simulink model "gtm_design_lpv"  (R2021b)
settings: Solver=VariableStepAuto  StartTime=0.0  StopTime=10  FixedStep=0.005  MaxStep=0.005  RelTol=1e-3
StopFcn:
  | MWSout=grabmws(bdroot);
  | MWSout.lastrun=datestr(now);
values from neighbouring files (symbols this model uses):
  s = tf('s')    [SingleDOF.m]    (also in main.m; mainSimple.m; newmain.m)
undefined symbols (not defined in the file or in its folder): Aero, aftfuel, aftfuel_pos, AILL, AILLC, AILR, AILRC, alpha_deg, altitude_ft, Ax_g, Ay_g, Az_g, b, beta_deg, bias, BRAKEC, Cbar, cg_pos0, cg_shift_gear, DamageCase, DamageModels, DamageOnsetTime, Earth, ELLIB, ELLIBC, ELLOB, ELLOBC, ELRIB, ELRIBC, ELROB, ELROBC, engl_ang, engl_pos, engr_ang, engr_pos, FLAPLIB, FLAPLIC, FLAPLOB, FLAPLOC, FLAPRIB, FLAPRIC, FLAPROB, FLAPROC, ft, FuelUsed_Init, fwdfuel, fwdfuel_pos, GEAR, GEARC, Inertia0, Inertia_shift_gear, Ixx_model, Iyy_model, Izz_model, KTAS, LandingGear, LengON, LinearizeModeOn, NAV_altitude_m, NAV_latitude_deg ... (+51)
libraries: simulink_extras x63, simulink_need_slupdate x30, LPVBlockLibrary x20, aerolibconvert2 x6, aerolibtransform2 x5, uavalgslib x4, UserContent_lib x3, simulink x3, robotcorelib x1, uavutilslib x1
(part 1 of 8)
settings Model: LastModifiedBy=jihoo
settings DataIOCC: ReturnWorkspaceOutputs=off
settings OptimizationCC: BlockReduction=off  BooleanDataType=off
settings DebuggingCC: SaveWithParameterizedLinksMsg=none  UnderspecifiedInitializationDetection=Classic  MergeDetectMultiDrivingBlocksExec=none  SignalResolutionControl=TryResolveAllWithWarning  InitInArrayFormatMsg=none
settings HardwareCC: TargetUnknown=on
settings ModelReferenceCC: PropagateSignalLabelsOutOfModel=off

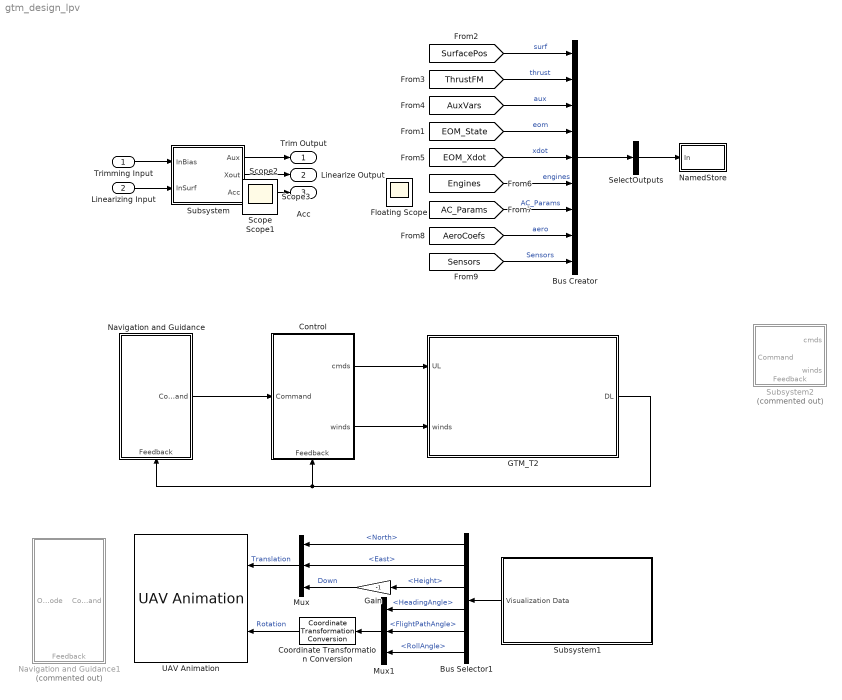
== system gtm_design_lpv ==
  Trimming Input : Inport  OutDataTypeStr=double  PortDimensions=4
  Linearizing Input : Inport  Port=2  OutDataTypeStr=double  PortDimensions=19
  Bus Creator : BusCreator  Inputs=9
  Bus Selector1 : BusSelector  OutputSignals=North,East,Height,HeadingAngle,FlightPathAngle,RollAngle
  Control : Subsystem
      settings: PortSchema="{\"entries\":[{\"content\":{\"sides\":[{\"content\":{\"connectorIds\":[\"In1\"]},\"type\":\"ConnectorPlacement.EquallySpacedRectSide\",\"uuid\":\"876f9d1c-31d1-4d48-8cbb-f6088518770e\"},{\"content\":{\"connectorIds\":[\"Out1\",\"Out2\"],\"side\":\"RIGHT\"},\"type\":\"ConnectorPlacement.EquallySpacedRectSide\",\"uuid\":\"0e4266e3-a031-465f-8381-066e8420e2a4\"},{\"content\":{\"connectorIds\":[],\"side\":\"TOP\"},\"type\":\"ConnectorPlacement.EquallySpacedRectSide\",\"uuid\":\"3957ab9c-ff96-432b-bd6f-14b7cf2f8092\"},{\"content\":{\"connectorIds\":[\"In2\"],\"side\":\"BOTTOM\"},\"type\":\"ConnectorPlacement.EquallySpacedRectSide\",\"uuid\":\"1e447cfa-7c82-4ae0-9a3c-28fe1a02d81e\"}]},\"type\":\"ConnectorPlacement.EquallySpacedConnector\",\"uuid\":\"5c345d19-69a3-46c5-b9cf-f35f763eae5c\"}],\"packageUris\":[\"http://schema.mathworks.com/mf0/Connector/R2020b\"],\"version\":\"1.0\"}"
  Coordinate Transformation Conversion : robotcorelib/Coordinate Transformation Conversion  InputRepresentation=Euler Angles  InputEulerSequence=ZYX  ShowTrVecInputPort=on  OutputRepresentation=Quaternion  OutputEulerSequence=ZYX  ShowTrVecOutputPort=on  SimulateUsing=Code generation
      settings: SourceProductBaseCode=NV,RO,RR,UV
  GTM_T2 : Subsystem  Tag=From trunk/GTMsim/gtm_model.mdl revision 162
      mask Display: image(imread('GTMtiny.png'))
  Gain : Gain  Gain=-1
  Mux : Mux  Inputs=3
  Mux1 : Mux  Inputs=3
  NamedStore : Subsystem  StopFcn=|  mask{enable_logging=on, do_stopfcn_callback=on}
      | % if strmatch(get_param(gcb,'do_stopfcn_callback'),...
      | % 'on','exact')                                       
      | %    if exist('logsout','var')                        
      | %        sout = CreateSimOut(logsout);                
      | %    else                                             
      | %         %disp('No Log Data Variable')               
      | %     end                                             
      | % clear logsout                                       
      | % end
      mask prompts: enable_logging "Enable Data Logging"; do_stopfcn_callback "Post-process logsout"
      mask help: Produces signal log of input data. If post processing is selected the logsout object is converted into a data structure (sout) with fields named after the bus signals. In this case a common time base is recommended.
      mask init:
      | H=get_param([gcb,'/In'],'PortHandles');
      | if (enable_logging)
      |     set(H.Outport(1),'DataLogging','on')
      | else
      |     set(H.Outport(1),'DataLogging','off')
      |     
      | end
  Navigation and Guidance : Subsystem
      settings: PortSchema="{\"entries\":[{\"content\":{\"sides\":[{\"content\":{\"connectorIds\":[]},\"type\":\"ConnectorPlacement.EquallySpacedRectSide\",\"uuid\":\"90854f57-5bb3-4250-804d-ac09ea809a44\"},{\"content\":{\"connectorIds\":[\"Out1\"],\"side\":\"RIGHT\"},\"type\":\"ConnectorPlacement.EquallySpacedRectSide\",\"uuid\":\"60962e56-1ad7-44d3-901b-e4e8a3eb3ce1\"},{\"content\":{\"connectorIds\":[],\"side\":\"TOP\"},\"type\":\"ConnectorPlacement.EquallySpacedRectSide\",\"uuid\":\"face4b20-fd55-46eb-98c2-63599aba0959\"},{\"content\":{\"connectorIds\":[\"In1\"],\"side\":\"BOTTOM\"},\"type\":\"ConnectorPlacement.EquallySpacedRectSide\",\"uuid\":\"a5d6b840-59da-4fbb-8659-3c66a691c6e0\"}]},\"type\":\"ConnectorPlacement.EquallySpacedConnector\",\"uuid\":\"30f94791-aa21-40a3-94e2-49d0efe50b10\"}],\"packageUris\":[\"http://schema.mathworks.com/mf0/Connector/R2020b\"],\"version\":\"1.0\"}"
  Navigation and Guidance1 : Subsystem  Commented=on
      settings: PortSchema="{\"entries\":[{\"content\":{\"sides\":[{\"content\":{\"connectorIds\":[\"In1\"]},\"type\":\"ConnectorPlacement.EquallySpacedRectSide\",\"uuid\":\"90854f57-5bb3-4250-804d-ac09ea809a44\"},{\"content\":{\"connectorIds\":[\"Out1\"],\"side\":\"RIGHT\"},\"type\":\"ConnectorPlacement.EquallySpacedRectSide\",\"uuid\":\"60962e56-1ad7-44d3-901b-e4e8a3eb3ce1\"},{\"content\":{\"connectorIds\":[],\"side\":\"TOP\"},\"type\":\"ConnectorPlacement.EquallySpacedRectSide\",\"uuid\":\"face4b20-fd55-46eb-98c2-63599aba0959\"},{\"content\":{\"connectorIds\":[\"In2\"],\"side\":\"BOTTOM\"},\"type\":\"ConnectorPlacement.EquallySpacedRectSide\",\"uuid\":\"a5d6b840-59da-4fbb-8659-3c66a691c6e0\"}]},\"type\":\"ConnectorPlacement.EquallySpacedConnector\",\"uuid\":\"30f94791-aa21-40a3-94e2-49d0efe50b10\"}],\"packageUris\":[\"http://schema.mathworks.com/mf0/Connector/R2020b\"],\"version\":\"1.0\"}"
  SelectOutputs : BusSelector  OutputSignals=surf,thrust,aux,eom,xdot,engines,AC_Params,aero,Sensors  OutputAsBus=on
  Subsystem : Subsystem
  Subsystem1 : Subsystem
  Subsystem2 : Subsystem  Commented=on
      settings: PortSchema="{\"entries\":[{\"content\":{\"sides\":[{\"content\":{\"connectorIds\":[\"In1\"]},\"type\":\"ConnectorPlacement.EquallySpacedRectSide\",\"uuid\":\"5c2295be-4c8d-43d5-89d0-a9519d1e786b\"},{\"content\":{\"connectorIds\":[\"Out1\",\"Out2\"],\"side\":\"RIGHT\"},\"type\":\"ConnectorPlacement.EquallySpacedRectSide\",\"uuid\":\"0338c219-9523-4a98-a604-936e4d0799a1\"},{\"content\":{\"connectorIds\":[],\"side\":\"TOP\"},\"type\":\"ConnectorPlacement.EquallySpacedRectSide\",\"uuid\":\"01cfcb74-d03a-4fe9-8f17-a2d3b8ee66f0\"},{\"content\":{\"connectorIds\":[\"In2\"],\"side\":\"BOTTOM\"},\"type\":\"ConnectorPlacement.EquallySpacedRectSide\",\"uuid\":\"93f21525-f5cf-4ae2-b844-2a7328abed77\"}]},\"type\":\"ConnectorPlacement.EquallySpacedConnector\",\"uuid\":\"4d608291-8d9a-4652-b4af-32d3e417625b\"}],\"packageUris\":[\"http://schema.mathworks.com/mf0/Connector/R2020b\"],\"version\":\"1.0\"}"
  UAV Animation : uavutilslib/UAV Animation  UAVType=FixedWing  UAVSize=50  InertialZDirection=Down  SampleTime=0.1
      settings: SourceProductBaseCode=UV
  Trim Output : Outport  OutDataTypeStr=double  PortDimensions=6
  Linearize Output : Outport  Port=2  OutDataTypeStr=double  PortDimensions=12
  Acc : Outport  Port=3  OutDataTypeStr=double  PortDimensions=3
  Floating Scope : Scope
  Scope{,1..3} (4 alike) : Scope
  wires:
  Linearizing Input/1 -> Subsystem/2(InSurf)
  Subsystem/1(Aux) -> Trim Output/1
  Subsystem/2(Xout) -> Linearize Output/1
  Trimming Input/1 -> Subsystem/1(InBias)
  Control/1(cmds) -> GTM_T2/1(UL)
  Control/2(winds) -> GTM_T2/2(winds)
  Subsystem/3(Acc) -> Acc/1
  Bus Selector1/6 -> Mux1/3  "<RollAngle>"
  Mux/1 -> UAV Animation/1  "Translation"
  Bus Selector1/2 -> Mux/2  "<East>"
  Mux1/1 -> Coordinate Transformation Conversion/1
  Bus Selector1/1 -> Mux/1  "<North>"
  Bus Selector1/4 -> Mux1/1  "<HeadingAngle>"
  Coordinate Transformation Conversion/1 -> UAV Animation/2  "Rotation"
  Bus Selector1/3 -> Gain/1  "<Height>"
  Bus Selector1/5 -> Mux1/2  "<FlightPathAngle>"
  Gain/1 -> Mux/3  "Down"
  GTM_T2/1(DL) -> Navigation and Guidance/1(Feedback), Control/2(Feedback)
  Navigation and Guidance/1(Command) -> Control/1(Command)
  Subsystem1/1(Visualization Data) -> Bus Selector1/1
  SelectOutputs/1 -> NamedStore/1(In)
  [AuxVars] -> Bus Creator/3  "aux"
  [ThrustFM] -> Bus Creator/2  "thrust"
  Bus Creator/1 -> SelectOutputs/1
  [SurfacePos] -> Bus Creator/1  "surf"
  [Sensors] -> Bus Creator/9  "Sensors"
  [Engines] -> Bus Creator/6  "engines"
  [EOM_Xdot] -> Bus Creator/5  "xdot"
  [AeroCoefs] -> Bus Creator/8  "aero"
  [AC_Params] -> Bus Creator/7  "AC_Params"
  [EOM_State] -> Bus Creator/4  "eom"

== system gtm_design_lpv/Control ==
  note: Input aileron command
      | +ail_cmd = roll left
  Command : Inport
  Feedback : Inport  Port=2
  Bus Creator : BusCreator  Inputs=21
  Bus Selector : BusSelector  OutputSignals=AirData.KTAS,AirData.altitude_ft
  Constant{1..4} (4 alike) : Constant  Value=0
  Demux : Demux
  Gain{1..21} (21 alike) : Gain  SaturateOnIntegerOverflow=on  OutDataTypeStr=Inherit: Same as input  ParamDataTypeStr=Inherit: Same as input
  Hinf : Subsystem  Commented=on  TreatAsAtomicUnit=on
  Input Generator : UserContent_lib/Input Generator  Commented=on  SystemSampleTime=-1  VariantActivationTime=update diagram  Latency=0  AutoFrameSizeCalculation=off
      link override Doublet Generator: timeon=[2 12 7]  pulsewidth=[0.5 0.5 0.5]  amplitude=[0 0 0]
  LPV : Subsystem  Commented=on  TreatAsAtomicUnit=on
  LPV1 : Subsystem  Commented=on  TreatAsAtomicUnit=on
  Left Roll Spoiler Schedule : Lookup  InputValues="[-20\t-11.76\t-2.36\t0\t2.36\t11.76\t20\t]"  Table=[0 0 0 0 0 9 45]  LookUpMeth=Interpolation-Use End Values
  Right Roll Spoiler Schedule : Lookup  InputValues="[-20\t-11.76\t-2.36\t0\t2.36\t11.76\t20\t]"  Table=[45 9 0 0 0 0 0]  LookUpMeth=Interpolation-Use End Values
  Scope1 : Scope  Commented=on
  Scope3 : Scope  Commented=on
  Scope4 : Scope  Commented=on
  Throttle Controller : Subsystem
  Winds : UserContent_lib/Input Generator/Winds  WindSpeed_knots=WindSpd  WindDirection_deg=WindDir  level=None
  cmds : Outport
  winds : Outport  Port=2
  wires:
  Constant1/1 -> Left Roll Spoiler Schedule/1, Right Roll Spoiler Schedule/1
  Left Roll Spoiler Schedule/1 -> Gain12/1, Gain13/1
  Gain9/1 -> Bus Creator/1  "THROTLC"
  Gain17/1 -> Bus Creator/16  "FLAPLOC"
  Gain5/1 -> Bus Creator/4  "ELLIBC"
  Gain20/1 -> Bus Creator/19  "GEARC"
  Gain11/1 -> Bus Creator/14  "SPLROBC"
  Gain8/1 -> Bus Creator/6  "ELRIBC"
  Gain13/1 -> Bus Creator/12  "SPLLOBC"
  Demux/4 -> Gain3/1, Gain4/1
  Gain1/1 -> Bus Creator/7  "AILLC"
  Demux/1 -> Gain8/1, Gain7/1, Gain5/1, Gain6/1
  Gain7/1 -> Bus Creator/5  "ELROBC"
  Gain15/1 -> Bus Creator/18  "FLAPROC"
  Constant4/1 -> Gain20/1
  Winds/1 -> winds/1
  Demux/3 -> Gain2/1
  Gain2/1 -> Bus Creator/8  "AILRC"
  Gain3/1 -> Bus Creator/9  "RUDUPC"
  Gain21/1 -> Bus Creator/21  "STEERC"
  Constant2/1 -> Gain15/1, Gain18/1, Gain17/1, Gain16/1
  Gain14/1 -> Bus Creator/13  "SPLRIBC"
  Constant3/1 -> Gain21/1, Gain19/1
  Gain6/1 -> Bus Creator/3  "ELLOBC"
  Right Roll Spoiler Schedule/1 -> Gain14/1, Gain11/1
  Gain10/1 -> Bus Creator/2  "THROTRC"
  Gain19/1 -> Bus Creator/20  "BRAKEC"
  Gain18/1 -> Bus Creator/17  "FLAPRIC"
  Gain4/1 -> Bus Creator/10  "RUDLOC"
  Bus Creator/1 -> cmds/1
  Bus Selector/2 -> Winds/2  "<altitude_ft>"
  Gain12/1 -> Bus Creator/11  "SPLLIBC"
  Gain16/1 -> Bus Creator/15  "FLAPLIC"
  Bus Selector/1 -> Winds/1  "<KTAS>"
  Throttle Controller/1(Out1) -> Gain9/1, Gain10/1
  Command/1 -> Hinf/1(Guidance), LPV1/1(Guidance), LPV/1(Guidance)
  Feedback/1 -> Bus Selector/1, LPV1/2(Feedback), Hinf/2(Feedback), LPV/2(Feedback)
  Demux/2 -> Gain1/1
  LPV/1(Out) -> Scope3/1
  LPV1/1(Out) -> Scope4/1
  Hinf/1(Out) -> Scope1/1
  ? -> Demux/1

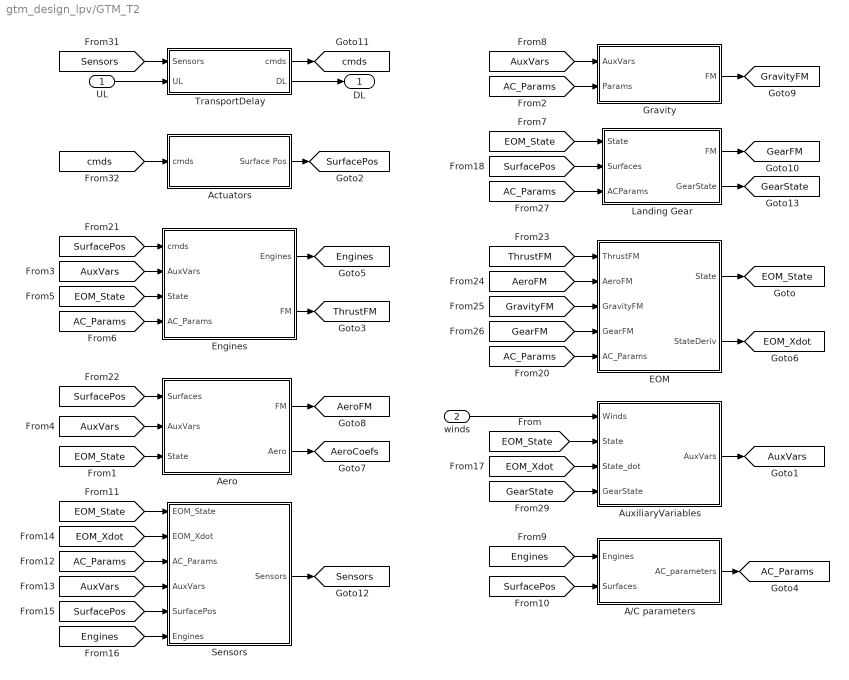
== system gtm_design_lpv/GTM_T2 ==
  UL : Inport
  winds : Inport  Port=2  PortDimensions=6
  A/C parameters : Subsystem
  Actuators : Subsystem
  Aero : Subsystem
  AuxiliaryVariables : Subsystem
  EOM : Subsystem
  Engines : Subsystem
  Gravity : Subsystem
  Landing Gear : Subsystem
  Sensors : Subsystem
  TransportDelay : Subsystem
  DL : Outport
  tag scope: AC_Params=global, AeroCoefs=global, AeroFM=global, AuxVars=global, EOM_State=global, EOM_Xdot=global, Engines=global, GearFM=global, GearState=global, GravityFM=global, Sensors=global, SurfacePos=global, ThrustFM=global, cmds=global
  wires:
  UL/1 -> TransportDelay/2(UL)
  TransportDelay/2(DL) -> DL/1
  Gravity/1(FM) -> [GravityFM]
  [AuxVars] -> Sensors/4(AuxVars)
  [EOM_Xdot] -> Sensors/2(EOM_Xdot)
  [Engines] -> Sensors/6(Engines)
  [SurfacePos] -> Sensors/5(SurfacePos)
  [AC_Params] -> Sensors/3(AC_Params)
  [EOM_State] -> Sensors/1(EOM_State)
  [AC_Params] -> EOM/5(AC_Params)
  [GearFM] -> EOM/4(GearFM)
  [GravityFM] -> EOM/3(GravityFM)
  [AeroFM] -> EOM/2(AeroFM)
  [ThrustFM] -> EOM/1(ThrustFM)
  [EOM_State] -> AuxiliaryVariables/2(State)
  [SurfacePos] -> Aero/1(Surfaces)
  [AC_Params] -> Landing Gear/3(ACParams)
  [SurfacePos] -> Engines/1(cmds)
  EOM/2(StateDeriv) -> [EOM_Xdot]
  [EOM_Xdot] -> AuxiliaryVariables/3(State_dot)
  Engines/1(Engines) -> [Engines]
  [SurfacePos] -> A/C parameters/2(Surfaces)
  [Engines] -> A/C parameters/1(Engines)
  A/C parameters/1(AC_parameters) -> [AC_Params]
  [AC_Params] -> Engines/4(AC_Params)
  [AuxVars] -> Engines/2(AuxVars)
  [EOM_State] -> Engines/3(State)
  [AuxVars] -> Gravity/1(AuxVars)
  [AC_Params] -> Gravity/2(Params)
  EOM/1(State) -> [EOM_State]
  Engines/2(FM) -> [ThrustFM]
  Aero/1(FM) -> [AeroFM]
  [AuxVars] -> Aero/2(AuxVars)
  AuxiliaryVariables/1(AuxVars) -> [AuxVars]
  [EOM_State] -> Aero/3(State)
  [EOM_State] -> Landing Gear/1(State)
  [SurfacePos] -> Landing Gear/2(Surfaces)
  Landing Gear/1(FM) -> [GearFM]
  Actuators/1(Surface Pos) -> [SurfacePos]
  winds/1 -> AuxiliaryVariables/1(Winds)
  TransportDelay/1(cmds) -> [cmds]
  [Sensors] -> TransportDelay/1(Sensors)
  [cmds] -> Actuators/1(cmds)
  Sensors/1(Sensors) -> [Sensors]
  Landing Gear/2(GearState) -> [GearState]
  [GearState] -> AuxiliaryVariables/4(GearState)
  Aero/2(Aero) -> [AeroCoefs]

== system gtm_design_lpv/NamedStore ==
  In : Inport
  Terminator : Terminator
  wires:
  In/1 -> Terminator/1  "SimOut"

== system gtm_design_lpv/Navigation and Guidance ==
  Feedback : Inport
  Bus Creator : BusCreator  Inputs=5
  Constant : Constant  Value=80
  Constant1 : Constant  Value=-12.5
  Demux : Demux  Outputs=3
  High-G Turn : Subsystem  Commented=on  TreatAsAtomicUnit=on
  Lateral Doublet : Subsystem  Commented=on  TreatAsAtomicUnit=on
  Longitudinal Doublet : Subsystem  TreatAsAtomicUnit=on
  Orbit Following : Subsystem  Commented=on  TreatAsAtomicUnit=on
  Pushover and Pullup : Subsystem  Commented=on  TreatAsAtomicUnit=on
  Scope : Scope
  Straight and Level Flight : Subsystem  Commented=on  TreatAsAtomicUnit=on
  Waypoint Following : Subsystem  Commented=on  TreatAsAtomicUnit=on
  Command : Outport
  wires:
  Bus Creator/1 -> Command/1
  Constant/1 -> Bus Creator/1  "V_c"
  Demux/1 -> Scope/1, Bus Creator/2  "An_c"
  Demux/2 -> Bus Creator/3  "beta_c"
  Demux/3 -> Bus Creator/4  "phi_c"
  Constant1/1 -> Bus Creator/5  "eta_sc"
  Feedback/1 -> Orbit Following/1(Feedback), Waypoint Following/1(Feedback)
  Longitudinal Doublet/1(Out1) -> Demux/1

== system gtm_design_lpv/Navigation and Guidance1 ==
  Operation Mode : Inport
  Feedback : Inport  Port=2
  Bus Creator : BusCreator  Inputs=5
  Constant : Constant  Value=80
  Constant1 : Constant  Value=-12.5
  Demux : Demux  Outputs=3
  High-G Turn : Subsystem  TreatAsAtomicUnit=on
  Lateral Doublet : Subsystem  TreatAsAtomicUnit=on
  Longitudinal Doublet : Subsystem  TreatAsAtomicUnit=on
  Merge : Merge  Inputs=7  InitialOutput=[1,0,0]
  Orbit Following : Subsystem  Commented=on  TreatAsAtomicUnit=on
  Pushover and Pullup : Subsystem  TreatAsAtomicUnit=on
  Straight and Level Flight : Subsystem  TreatAsAtomicUnit=on
  Switch Case2 : SwitchCase  CaseConditions={1,2,3,4,5,6}
  Waypoint Following : Subsystem  Commented=on  TreatAsAtomicUnit=on
  Command : Outport
  wires:
  Bus Creator/1 -> Command/1
  Constant/1 -> Bus Creator/1  "V_c"
  Demux/1 -> Bus Creator/2  "An_c"
  Demux/2 -> Bus Creator/3  "beta_c"
  Demux/3 -> Bus Creator/4  "phi_c"
  Constant1/1 -> Bus Creator/5  "eta_sc"
  Operation Mode/1 -> Switch Case2/1
  Feedback/1 -> Orbit Following/1(Feedback), Waypoint Following/1(Feedback)
  Longitudinal Doublet/1(Out1) -> Merge/1
  Lateral Doublet/1(Out1) -> Merge/2
  Straight and Level Flight/1(Out1) -> Merge/7
  Waypoint Following/1(Out1) -> Merge/5
  Merge/1 -> Demux/1
  Pushover and Pullup/1(Out1) -> Merge/3
  High-G Turn/1(Out1) -> Merge/4
  Orbit Following/1(Out1) -> Merge/6
  Switch Case2/1 -> Longitudinal Doublet/Action
  Switch Case2/2 -> Lateral Doublet/Action
  Switch Case2/3 -> Pushover and Pullup/Action
  Switch Case2/4 -> High-G Turn/Action
  Switch Case2/5 -> Waypoint Following/Action
  Switch Case2/6 -> Orbit Following/Action
  Switch Case2/7 -> Straight and Level Flight/Action

== system gtm_design_lpv/Subsystem ==
  InBias : Inport
  InSurf : Inport  Port=2
  Bus Selector : BusSelector  OutputSignals=eas,tas,alpha,beta,gamma,gndtrack  OutputAsBus=on
  Bus Selector1 : BusSelector  OutputSignals=Ax,Ay,Az  OutputAsBus=on
  Bus to Vector : BusToVector
  Bus to Vector1 : BusToVector
  Bus to Vector2 : BusToVector
  DocBlock : simulink/Model-Wide Utilities/DocBlock  DocumentType=Text
      content=|
      | Inputs and Outputs selected here have a specific ordering.
      |
      |
      |
      | Do not change this without also changing output channel ordering in associated linmodel.m and
      | trimgtm.m functions
  Aux : Outport
  Xout : Outport  Port=2
  Acc : Outport  Port=3
  tag scope: SurfaceBias=global, SurfaceDeltas=global
  wires:
  [EOM_State] -> Bus to Vector1/1  "eom"
  Bus Selector/1 -> Bus to Vector/1
  InSurf/1 -> [SurfaceDeltas]
  Bus to Vector/1 -> Aux/1
  Bus to Vector1/1 -> Xout/1
  InBias/1 -> [SurfaceBias]
  Bus to Vector2/1 -> Acc/1
  Bus Selector1/1 -> Bus to Vector2/1
  [AuxVars] -> Bus Selector1/1, Bus Selector/1  "aux"

== system gtm_design_lpv/Subsystem1 ==
  Bus Creator1 : BusCreator  Inputs=6
  Bus Selector1 : BusSelector  OutputSignals=latitude,longitude,altitude
  Bus Selector2 : BusSelector  OutputSignals=gndtrack,gamma
  Bus Selector3 : BusSelector  OutputSignals=phi
  Constant1 : Constant  Value=[37.827926944;-75.494061666]
  Constant2 : Constant  Value=0
  Constant3 : Constant  Value=0
  Degrees to Radians1 : simulink_extras/Transformations/Degrees to Radians
  Degrees to Radians2 : simulink_extras/Transformations/Degrees to Radians
  Demux1 : Demux  Outputs=3
      settings: DisplayOption=none
  Demux3 : Demux  Outputs=3
      settings: DisplayOption=none
  Display : Display
  Display1 : Display
  Gain : Gain  Gain=-1
  LLA to Flat Earth : aerolibtransform2/LLA to Flat Earth  units=English  ptype=Earth (WGS84)  F=1/298.257223563  R=20925646.3255  refPosPort=on  LL0=[0 10]  psi=0
      settings: SourceProductBaseCode=AE
  Mux : Mux  Inputs=3
  Mux2 : Mux  Inputs=2
  Radians to Degrees : simulink_extras/Transformations/Radians to Degrees
  Radians to Degrees1 : simulink_extras/Transformations/Radians to Degrees
  Scope : Scope
  To Workspace : ToWorkspace  VariableName=NED  SampleTime=-1
  Visualization Data : Outport
  wires:
  Demux1/3 -> Gain/1  "Down"
  Demux3/3 -> Bus Creator1/6  "RollAngle"
  Demux1/2 -> Bus Creator1/2  "East"
  Demux3/1 -> Bus Creator1/4  "HeadingAngle"
  Demux1/1 -> Bus Creator1/1  "North"
  Demux3/2 -> Bus Creator1/5  "FlightPathAngle"
  Bus Creator1/1 -> Visualization Data/1
  [EOM_State] -> Bus Selector1/1
  Gain/1 -> Bus Creator1/3  "Height"
  Bus Selector3/1 -> Mux/3  "<phi>"
  Degrees to Radians1/1 -> Mux/2  "gamma_rad"
  Degrees to Radians2/1 -> Mux/1  "gndtrack_rad"
  Mux/1 -> Demux3/1
  Constant3/1 -> LLA to Flat Earth/3
  Constant1/1 -> LLA to Flat Earth/4
  Constant2/1 -> LLA to Flat Earth/5
  Mux2/1 -> Display/1, LLA to Flat Earth/1
  Bus Selector1/3 -> Display1/1, LLA to Flat Earth/2  "<altitude>"
  [EOM_State] -> Bus Selector3/1  "eom"
  [AuxVars] -> Bus Selector2/1  "aux"
  Bus Selector2/1 -> Degrees to Radians2/1  "<gndtrack>"
  Bus Selector2/2 -> Degrees to Radians1/1  "<gamma>"
  Radians to Degrees/1 -> Mux2/1
  Radians to Degrees1/1 -> Mux2/2
  Bus Selector1/1 -> Radians to Degrees/1  "<latitude>"
  Bus Selector1/2 -> Radians to Degrees1/1  "<longitude>"
  LLA to Flat Earth/1 -> Demux1/1, To Workspace/1, Scope/1

== system gtm_design_lpv/Subsystem2 ==
  note: Input aileron command
      | +ail_cmd = roll left
  Command : Inport
  Feedback : Inport  Port=2
  Bus Creator : BusCreator  Inputs=21
  Bus Selector : BusSelector  OutputSignals=AirData.KTAS,AirData.altitude_ft
  Constant : Constant  Value=0.01
  Constant{1..4} (4 alike) : Constant  Value=0
  Demux : Demux
  Gain{1..21} (21 alike) : Gain  SaturateOnIntegerOverflow=on  OutDataTypeStr=Inherit: Same as input  ParamDataTypeStr=Inherit: Same as input
  Hinf : Subsystem  Commented=on  TreatAsAtomicUnit=on
  LPV : Subsystem  TreatAsAtomicUnit=on
  LPV1 : Subsystem  Commented=on  TreatAsAtomicUnit=on
  Left Roll Spoiler Schedule : Lookup  InputValues="[-20\t-11.76\t-2.36\t0\t2.36\t11.76\t20\t]"  Table=[0 0 0 0 0 9 45]  LookUpMeth=Interpolation-Use End Values
  Right Roll Spoiler Schedule : Lookup  InputValues="[-20\t-11.76\t-2.36\t0\t2.36\t11.76\t20\t]"  Table=[45 9 0 0 0 0 0]  LookUpMeth=Interpolation-Use End Values
  Scope1 : Scope  Commented=on
  Scope3 : Scope
  Scope4 : Scope  Commented=on
  Throttle Controller : Subsystem
  Winds : UserContent_lib/Input Generator/Winds  WindSpeed_knots=WindSpd  WindDirection_deg=WindDir  level=None
  cmds : Outport
  winds : Outport  Port=2
  wires:
  Hinf/1(Out) -> Scope1/1
  LPV/1(Out) -> Scope3/1
  LPV1/1(Out) -> Scope4/1
  Feedback/1 -> Bus Selector/1, LPV1/2(Feedback), Hinf/2(Feedback), LPV/2(Feedback)
  Winds/1 -> winds/1
  Bus Selector/1 -> Winds/1  "<KTAS>"
  Bus Selector/2 -> Winds/2  "<altitude_ft>"
  Command/1 -> Hinf/1(Guidance), LPV1/1(Guidance), LPV/1(Guidance)
  Demux/2 -> Gain1/1
  Gain21/1 -> Bus Creator/21  "STEERC"
  Gain4/1 -> Bus Creator/10  "RUDLOC"
  Demux/1 -> Gain8/1, Gain7/1, Gain5/1, Gain6/1
  Constant3/1 -> Gain21/1, Gain19/1
  Gain16/1 -> Bus Creator/15  "FLAPLIC"
  Constant2/1 -> Gain15/1, Gain18/1, Gain17/1, Gain16/1
  Gain13/1 -> Bus Creator/12  "SPLLOBC"
  Demux/3 -> Gain2/1
  Gain8/1 -> Bus Creator/6  "ELRIBC"
  Demux/4 -> Gain3/1, Gain4/1
  Gain15/1 -> Bus Creator/18  "FLAPROC"
  Gain3/1 -> Bus Creator/9  "RUDUPC"
  Gain12/1 -> Bus Creator/11  "SPLLIBC"
  Gain2/1 -> Bus Creator/8  "AILRC"
  Gain18/1 -> Bus Creator/17  "FLAPRIC"
  Gain11/1 -> Bus Creator/14  "SPLROBC"
  Right Roll Spoiler Schedule/1 -> Gain14/1, Gain11/1
  Gain17/1 -> Bus Creator/16  "FLAPLOC"
  Gain10/1 -> Bus Creator/2  "THROTRC"
  Constant4/1 -> Gain20/1
  Gain1/1 -> Bus Creator/7  "AILLC"
  Gain19/1 -> Bus Creator/20  "BRAKEC"
  Gain6/1 -> Bus Creator/3  "ELLOBC"
  Gain7/1 -> Bus Creator/5  "ELROBC"
  Gain20/1 -> Bus Creator/19  "GEARC"
  Left Roll Spoiler Schedule/1 -> Gain12/1, Gain13/1
  Constant1/1 -> Left Roll Spoiler Schedule/1, Right Roll Spoiler Schedule/1
  Gain14/1 -> Bus Creator/13  "SPLRIBC"
  Gain5/1 -> Bus Creator/4  "ELLIBC"
  Bus Creator/1 -> cmds/1
  Throttle Controller/1(Out1) -> Gain10/1, Gain9/1
  Gain9/1 -> Bus Creator/1  "THROTLC"
  Constant/1 -> Demux/1

== system gtm_design_lpv/Control/Hinf ==
  Guidance : Inport
  Feedback : Inport  Port=2
  Add : Sum
  Bus Selector : BusSelector  OutputSignals=AirData.KTAS,AirData.altitude_ft,SurfacePos.AILL,SurfacePos.AILR
  Bus Selector3 : BusSelector  OutputSignals=An_c
  Bus Selector4 : BusSelector  OutputSignals=beta_c,phi_c  OutputAsBus=on
  Bus Selector5 : BusSelector  OutputSignals=AirData.alpha_deg,MAG3.q_deg,MAG3.Az_g
  Bus Selector6 : BusSelector  OutputSignals=AirData.beta_deg,MAG3.p_deg,MAG3.r_deg,MIDG.phi_deg,MAG3.Ay_g
  Bus to Vector : BusToVector
  Bus to Vector1 : BusToVector
  Constant : Constant
  Degrees to Radians{,1..5} (6 alike) : simulink_extras/Transformations/Degrees to Radians
  Demux1 : Demux  Outputs=2
  Gain : Gain  Gain=1/2
  Gain1 : Gain  Gain=1/100
  Gain2 : Gain  Gain=32.17405
  Gain3 : Gain  Gain=32.17405
  Gain4 : Gain  Gain=100
  Gain5 : Gain  Gain=100
  LPVBlock1 : LPVBlockLibrary/LPVBlock  sys=K_lon_hinf  plist={'rho1_tas_param';'rho2_alt_param';'rho3_mor_param'}  x0=0
      settings: SourceProductName=LPVTools Blocks
  LPVBlock2 : LPVBlockLibrary/LPVBlock  sys=K_lat_hinf  plist={'rho1_tas_param';'rho2_alt_param';'rho3_mor_param'}  x0=0
      settings: SourceProductName=LPVTools Blocks
  LPVBlock3 : LPVBlockLibrary/LPVBlock  sys=sch_alp_trim  plist={'rho1_tas_param';'rho2_alt_param';'rho3_mor_param'}  x0=0
      settings: SourceProductName=LPVTools Blocks
  Mux : Mux  Inputs=3
  Mux5 : Mux  Inputs=[1 1 1 1]
  Mux6 : Mux  Inputs=5
  Mux7 : Mux  Inputs=2
  Mux8 : Mux
  Radians to Degrees : simulink_extras/Transformations/Radians to Degrees
  Radians to Degrees1 : simulink_extras/Transformations/Radians to Degrees
  Selector : Selector  InputPortWidth=3  IndexOptions=Index vector (dialog)  Indices=3  OutputSizes=1
  Sum : Sum  Inputs=|+-
  Sum1 : Sum  Inputs=++|
  Sum2 : Sum  Inputs=|+-
  Out : Outport  InitialOutput=zeros(4,1)
  wires:
  Bus to Vector/1 -> Mux7/1
  Bus Selector4/1 -> Bus to Vector/1
  Bus to Vector1/1 -> Mux5/1
  Bus Selector3/1 -> Bus to Vector1/1  "<An_c>"
  Mux5/1 -> LPVBlock1/1
  Degrees to Radians/1 -> Mux5/2
  Degrees to Radians1/1 -> Mux5/3
  Gain2/1 -> Mux5/4
  Mux8/1 -> Out/1
  Radians to Degrees1/1 -> Mux8/1
  Gain4/1 -> Mux8/2
  Gain5/1 -> Mux8/3
  Radians to Degrees/1 -> Mux8/4
  Demux1/2 -> Radians to Degrees/1
  Sum1/1 -> Gain5/1
  Sum2/1 -> Gain4/1
  Demux1/1 -> Sum2/1, Sum1/2
  Selector/1 -> Sum2/2, Sum1/1
  [rho] -> Selector/1
  LPVBlock1/1 -> Radians to Degrees1/1
  LPVBlock2/1 -> Demux1/1
  [rho] -> LPVBlock2/2
  Mux7/1 -> LPVBlock2/1
  Mux6/1 -> Mux7/2
  Degrees to Radians5/1 -> Mux6/4
  Degrees to Radians4/1 -> Mux6/3
  Degrees to Radians3/1 -> Mux6/2
  Degrees to Radians2/1 -> Mux6/1
  Gain3/1 -> Mux6/5
  Bus Selector6/5 -> Gain3/1  "<Ay_g>"
  Bus Selector6/4 -> Degrees to Radians5/1  "<phi_deg>"
  Bus Selector6/3 -> Degrees to Radians4/1  "<r_deg>"
  Bus Selector6/2 -> Degrees to Radians3/1  "<p_deg>"
  Bus Selector6/1 -> Degrees to Radians2/1  "<beta_deg>"
  Sum/1 -> Degrees to Radians/1
  LPVBlock3/1 -> Sum/2
  Bus Selector5/2 -> Degrees to Radians1/1  "<q_deg>"
  [rho] -> LPVBlock3/2
  Constant/1 -> LPVBlock3/1
  [rho] -> LPVBlock1/2
  Bus Selector5/3 -> Gain2/1  "<Az_g>"
  Bus Selector5/1 -> Sum/1  "<alpha_deg>"
  Guidance/1 -> Bus Selector3/1, Bus Selector4/1
  Gain1/1 -> Mux/3
  Add/1 -> Gain/1
  Feedback/1 -> Bus Selector5/1, Bus Selector6/1, Bus Selector/1
  Bus Selector/1 -> Mux/1  "<KTAS>"
  Bus Selector/3 -> Add/1  "<AILL>"
  Bus Selector/4 -> Add/2  "<AILR>"
  Bus Selector/2 -> Mux/2  "<altitude_ft>"
  Gain/1 -> Gain1/1
  Mux/1 -> [rho]

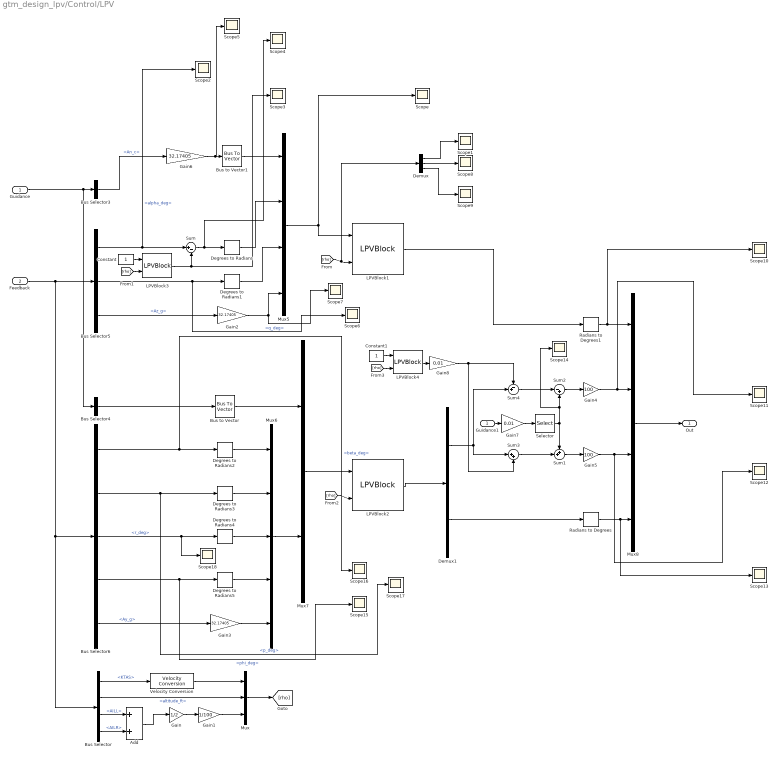
== system gtm_design_lpv/Control/LPV ==
  Guidance : Inport
  Feedback : Inport  Port=2
  Add : Sum
  Bus Selector : BusSelector  OutputSignals=AirData.KTAS,AirData.altitude_ft,SurfacePos.AILL,SurfacePos.AILR
  Bus Selector3 : BusSelector  OutputSignals=An_c
  Bus Selector4 : BusSelector  OutputSignals=beta_c,phi_c  OutputAsBus=on
  Bus Selector5 : BusSelector  OutputSignals=AirData.alpha_deg,MAG3.q_deg,MAG3.Az_g
  Bus Selector6 : BusSelector  OutputSignals=AirData.beta_deg,MAG3.p_deg,MAG3.r_deg,MIDG.phi_deg,MAG3.Ay_g
  Bus to Vector : BusToVector
  Bus to Vector1 : BusToVector
  Constant : Constant
  Constant1 : Constant
  Degrees to Radians{,1..5} (6 alike) : simulink_extras/Transformations/Degrees to Radians
  Demux : Demux  Outputs=3
  Demux1 : Demux  Outputs=2
  Gain : Gain  Gain=1/2
  Gain1 : Gain  Gain=1/100
  Gain2 : Gain  Gain=32.17405
  Gain3 : Gain  Gain=32.17405
  Gain4 : Gain  Gain=100
  Gain5 : Gain  Gain=100
  Gain6 : Gain  Gain=32.17405
  Gain7 : Gain  Gain=0.01
  Gain8 : Gain  Gain=0.01
  Guidance1 : InportShadow
  LPVBlock1 : LPVBlockLibrary/LPVBlock  sys=K_lon_lpv  plist={'rho1_tas_param';'rho2_alt_param';'rho3_mor_param'}  x0=0
      settings: SourceProductName=LPVTools Blocks
  LPVBlock2 : LPVBlockLibrary/LPVBlock  sys=K_lat_lpv  plist={'rho1_tas_param';'rho2_alt_param';'rho3_mor_param'}  x0=0
      settings: SourceProductName=LPVTools Blocks
  LPVBlock3 : LPVBlockLibrary/LPVBlock  sys=sch_alp_trim  plist={'rho1_tas_param';'rho2_alt_param';'rho3_mor_param'}  x0=0
      settings: SourceProductName=LPVTools Blocks
  LPVBlock4 : LPVBlockLibrary/LPVBlock  sys=sch_aileron_trim  plist={'rho1_tas_param';'rho2_alt_param';'rho3_mor_param'}  x0=0
      settings: SourceProductName=LPVTools Blocks
  Mux : Mux  Inputs=3
  Mux5 : Mux  Inputs=[1 1 1 1]
  Mux6 : Mux  Inputs=5
  Mux7 : Mux  Inputs=2
  Mux8 : Mux
  Radians to Degrees : simulink_extras/Transformations/Radians to Degrees
  Radians to Degrees1 : simulink_extras/Transformations/Radians to Degrees
  Scope{,1..18} (19 alike) : Scope
  Selector : Selector  InputPortWidth=5  IndexOptions=Index vector (dialog)  Indices=5  OutputSizes=1
  Sum : Sum  Inputs=|+-
  Sum1 : Sum  Inputs=++|
  Sum2 : Sum  Inputs=|-+
  Sum3 : Sum  Inputs=|++
  Sum4 : Sum  Inputs=-+|
  Velocity Conversion : aerolibconvert2/Velocity Conversion  IU=kts  OU=ft/s
  Out : Outport  InitialOutput=zeros(4,1)
  wires:
  Mux/1 -> [rho]
  Gain/1 -> Gain1/1
  Bus Selector/2 -> Mux/2  "<altitude_ft>"
  Bus Selector/4 -> Add/2  "<AILR>"
  Bus Selector/3 -> Add/1  "<AILL>"
  Bus Selector/1 -> Velocity Conversion/1  "<KTAS>"
  Feedback/1 -> Bus Selector/1, Bus Selector6/1, Bus Selector5/1
  Add/1 -> Gain/1
  Gain1/1 -> Mux/3
  Guidance/1 -> Bus Selector4/1, Bus Selector3/1
  Bus Selector5/1 -> Scope2/1, Sum/1  "<alpha_deg>"
  Bus Selector5/3 -> Gain2/1  "<Az_g>"
  [rho] -> Demux/1, LPVBlock1/2
  Constant/1 -> LPVBlock3/1
  [rho] -> LPVBlock3/2
  Bus Selector5/2 -> Scope6/1, Degrees to Radians1/1  "<q_deg>"
  LPVBlock3/1 -> Scope3/1, Sum/2
  Sum/1 -> Scope4/1, Degrees to Radians/1
  Bus Selector6/1 -> Scope16/1, Degrees to Radians2/1  "<beta_deg>"
  Bus Selector6/2 -> Scope17/1, Degrees to Radians3/1  "<p_deg>"
  Bus Selector6/3 -> Scope18/1, Degrees to Radians4/1  "<r_deg>"
  Bus Selector6/4 -> Scope15/1, Degrees to Radians5/1  "<phi_deg>"
  Bus Selector6/5 -> Gain3/1  "<Ay_g>"
  Gain3/1 -> Mux6/5
  Degrees to Radians2/1 -> Mux6/1
  Degrees to Radians3/1 -> Mux6/2
  Degrees to Radians4/1 -> Mux6/3
  Degrees to Radians5/1 -> Mux6/4
  Mux6/1 -> Mux7/2
  Mux7/1 -> LPVBlock2/1
  [rho] -> LPVBlock2/2
  LPVBlock2/1 -> Demux1/1
  LPVBlock1/1 -> Radians to Degrees1/1
  Selector/1 -> Sum1/1, Scope14/1, Sum2/2
  Demux1/1 -> Sum3/1, Sum4/2
  Sum2/1 -> Gain4/1
  Sum1/1 -> Gain5/1
  Demux1/2 -> Radians to Degrees/1
  Radians to Degrees/1 -> Scope13/1, Mux8/4
  Gain5/1 -> Scope12/1, Mux8/3
  Gain4/1 -> Scope11/1, Mux8/2
  Radians to Degrees1/1 -> Scope10/1, Mux8/1
  Mux8/1 -> Out/1
  Gain2/1 -> Mux5/4, Scope7/1
  Degrees to Radians1/1 -> Mux5/3
  Degrees to Radians/1 -> Mux5/2
  Mux5/1 -> LPVBlock1/1, Scope/1
  Bus Selector3/1 -> Gain6/1  "<An_c>"
  Bus to Vector1/1 -> Mux5/1
  Bus Selector4/1 -> Bus to Vector/1
  Bus to Vector/1 -> Mux7/1
  Velocity Conversion/1 -> Mux/1
  Demux/2 -> Scope8/1
  Demux/1 -> Scope1/1
  Demux/3 -> Scope9/1
  Gain6/1 -> Scope5/1, Bus to Vector1/1
  Guidance1/1 -> Gain7/1
  Gain7/1 -> Selector/1
  Constant1/1 -> LPVBlock4/1
  [rho] -> LPVBlock4/2
  Sum4/1 -> Sum2/1
  Sum3/1 -> Sum1/2
  Gain8/1 -> Sum4/1, Sum3/2
  LPVBlock4/1 -> Gain8/1

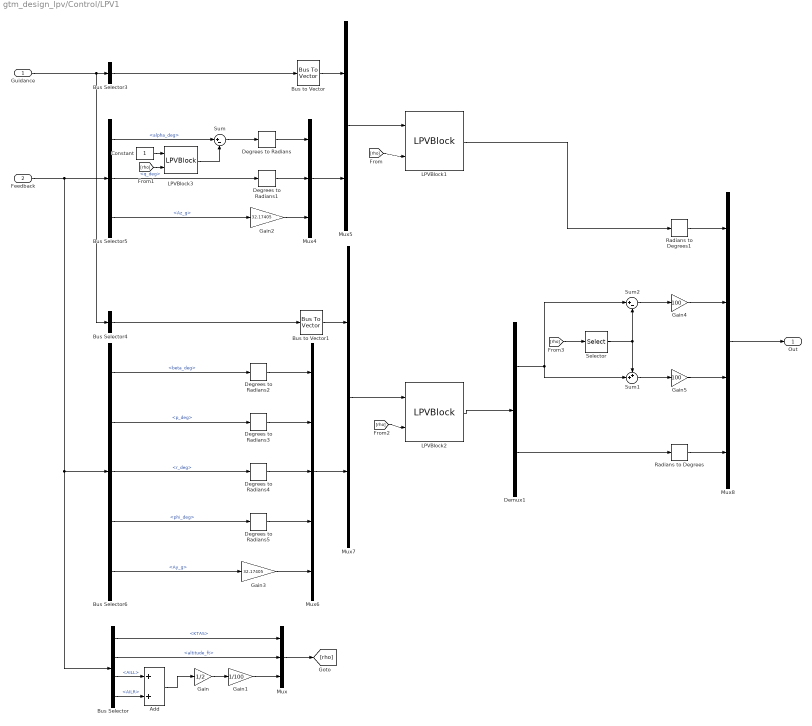
== system gtm_design_lpv/Control/LPV1 ==
  Guidance : Inport
  Feedback : Inport  Port=2
  Add : Sum
  Bus Selector : BusSelector  OutputSignals=AirData.KTAS,AirData.altitude_ft,SurfacePos.AILL,SurfacePos.AILR
  Bus Selector3 : BusSelector  OutputSignals=An_c  OutputAsBus=on
  Bus Selector4 : BusSelector  OutputSignals=beta_c,phi_c  OutputAsBus=on
  Bus Selector5 : BusSelector  OutputSignals=AirData.alpha_deg,MAG3.q_deg,MAG3.Az_g
  Bus Selector6 : BusSelector  OutputSignals=AirData.beta_deg,MAG3.p_deg,MAG3.r_deg,MIDG.phi_deg,MAG3.Ay_g
  Bus to Vector : BusToVector
  Bus to Vector1 : BusToVector
  Constant : Constant
  Degrees to Radians{,1..5} (6 alike) : simulink_extras/Transformations/Degrees to Radians
  Demux1 : Demux  Outputs=2
  Gain : Gain  Gain=1/2
  Gain1 : Gain  Gain=1/100
  Gain2 : Gain  Gain=32.17405
  Gain3 : Gain  Gain=32.17405
  Gain4 : Gain  Gain=100
  Gain5 : Gain  Gain=100
  LPVBlock1 : LPVBlockLibrary/LPVBlock  sys=K_lon_lpv  plist={'rho1_tas_param';'rho2_alt_param';'rho3_mor_param'}  x0=0
      settings: SourceProductName=LPVTools Blocks
  LPVBlock2 : LPVBlockLibrary/LPVBlock  sys=K_lat_lpv  plist={'rho1_tas_param';'rho2_alt_param';'rho3_mor_param'}  x0=0
      settings: SourceProductName=LPVTools Blocks
  LPVBlock3 : LPVBlockLibrary/LPVBlock  sys=sch_alp_trim  plist={'rho1_tas_param';'rho2_alt_param';'rho3_mor_param'}  x0=0
      settings: SourceProductName=LPVTools Blocks
  Mux : Mux  Inputs=3
  Mux4 : Mux  Inputs=3
  Mux5 : Mux  Inputs=2
  Mux6 : Mux  Inputs=5
  Mux7 : Mux  Inputs=2
  Mux8 : Mux
  Radians to Degrees : simulink_extras/Transformations/Radians to Degrees
  Radians to Degrees1 : simulink_extras/Transformations/Radians to Degrees
  Selector : Selector  InputPortWidth=3  IndexOptions=Index vector (dialog)  Indices=3  OutputSizes=1
  Sum : Sum  Inputs=|+-
  Sum1 : Sum  Inputs=++|
  Sum2 : Sum  Inputs=|+-
  Out : Outport  InitialOutput=zeros(4,1)
  wires:
  Mux8/1 -> Out/1
  Radians to Degrees1/1 -> Mux8/1
  Gain4/1 -> Mux8/2
  Gain5/1 -> Mux8/3
  Radians to Degrees/1 -> Mux8/4
  Demux1/2 -> Radians to Degrees/1
  Sum1/1 -> Gain5/1
  Sum2/1 -> Gain4/1
  Demux1/1 -> Sum2/1, Sum1/2
  Selector/1 -> Sum2/2, Sum1/1
  [rho] -> Selector/1
  LPVBlock1/1 -> Radians to Degrees1/1
  LPVBlock2/1 -> Demux1/1
  [rho] -> LPVBlock2/2
  Mux7/1 -> LPVBlock2/1
  Bus to Vector1/1 -> Mux7/1
  Mux6/1 -> Mux7/2
  Degrees to Radians5/1 -> Mux6/4
  Degrees to Radians4/1 -> Mux6/3
  Degrees to Radians3/1 -> Mux6/2
  Degrees to Radians2/1 -> Mux6/1
  Gain3/1 -> Mux6/5
  Bus Selector6/5 -> Gain3/1  "<Ay_g>"
  Bus Selector6/4 -> Degrees to Radians5/1  "<phi_deg>"
  Bus Selector6/3 -> Degrees to Radians4/1  "<r_deg>"
  Bus Selector6/2 -> Degrees to Radians3/1  "<p_deg>"
  Bus Selector6/1 -> Degrees to Radians2/1  "<beta_deg>"
  Gain2/1 -> Mux4/3
  Degrees to Radians1/1 -> Mux4/2
  Degrees to Radians/1 -> Mux4/1
  Sum/1 -> Degrees to Radians/1
  LPVBlock3/1 -> Sum/2
  Bus Selector5/2 -> Degrees to Radians1/1  "<q_deg>"
  [rho] -> LPVBlock3/2
  Constant/1 -> LPVBlock3/1
  [rho] -> LPVBlock1/2
  Mux5/1 -> LPVBlock1/1
  Bus to Vector/1 -> Mux5/1
  Mux4/1 -> Mux5/2
  Bus Selector5/3 -> Gain2/1  "<Az_g>"
  Bus Selector5/1 -> Sum/1  "<alpha_deg>"
  Bus Selector4/1 -> Bus to Vector1/1
  Bus Selector3/1 -> Bus to Vector/1
  Guidance/1 -> Bus Selector3/1, Bus Selector4/1
  Gain1/1 -> Mux/3
  Add/1 -> Gain/1
  Feedback/1 -> Bus Selector5/1, Bus Selector6/1, Bus Selector/1
  Bus Selector/1 -> Mux/1  "<KTAS>"
  Bus Selector/3 -> Add/1  "<AILL>"
  Bus Selector/4 -> Add/2  "<AILR>"
  Bus Selector/2 -> Mux/2  "<altitude_ft>"
  Gain/1 -> Gain1/1
  Mux/1 -> [rho]

== system gtm_design_lpv/Control/Throttle Controller ==
  Constant : Constant  Value=36.739425746701627
  Constant1 : Constant  Value=0
  Out1 : Outport
  wires:
  Constant1/1 -> Out1/1

== system gtm_design_lpv/GTM_T2/A//C parameters ==
  Engines : Inport
  Surfaces : Inport  Port=2
  B : Constant  Value=b
  Bus Creator4 : BusCreator  Inputs=15
  Bus Selector : BusSelector  OutputSignals=fuel_used
  Bus Selector1 : BusSelector  OutputSignals=GEAR
  Cbar : Constant  Value=Cbar
  Demux : Demux  Outputs=6
  Inertia/Mass/CG Shift : Subsystem  mask{DamageModels=DamageModels}
      mask prompts: DamageModels "Array of Damage Cases"
      mask init:
      | Ncases=length(DamageModels);
      | dCGDamage=zeros(Ncases+1,3);   
      | dMassDamage=zeros(Ncases+1,1);
      | dInertiaDamage=zeros(Ncases+1,6);
      | for i=1:Ncases,
      |   if isfield(DamageModels{i},'Mass'),
      |      dInertiaDamage(i+1,:)=DamageModels{i}.Mass.dIxxIyyIzzIxzIyzIxy;
      |      dCGDamage(i+1,:)=DamageModels{i}.Mass.dCG;
      |      dMassDamage(i+1)=DamageModels{i}.Mass.dWeight;
      |   end
      | end
  S : Constant  Value=S
  TriggerDamage : Subsystem
  ixxb5 : Constant  Value=engr_pos
  ixxb6 : Constant  Value=engl_pos
  xCG1 : Constant  Value=ref_cg
  AC_parameters : Outport
  wires:
  Bus Selector/1 -> Inertia/Mass/CG Shift/2(fuel_used)  "<fuel_used>"
  Bus Selector1/1 -> Inertia/Mass/CG Shift/1(gear)  "<GEAR>"
  [DamageCase] -> Inertia/Mass/CG Shift/3(DamageCase)
  [DamageCase] -> Bus Creator4/13  "DamageCase"
  Inertia/Mass/CG Shift/3(CG) -> Bus Creator4/12  "CG"
  Inertia/Mass/CG Shift/2(mass) -> Bus Creator4/11  "mass"
  Demux/6 -> Bus Creator4/10  "Ixy"
  Demux/5 -> Bus Creator4/9  "Iyz"
  Demux/4 -> Bus Creator4/8  "Ixz"
  Demux/3 -> Bus Creator4/7  "Izz"
  Demux/2 -> Bus Creator4/6  "Iyy"
  Demux/1 -> Bus Creator4/5  "Ixx"
  ixxb6/1 -> Bus Creator4/15  "LfEng"
  ixxb5/1 -> Bus Creator4/14  "RtEng"
  xCG1/1 -> Bus Creator4/4  "CP"
  B/1 -> Bus Creator4/3  "B"
  Cbar/1 -> Bus Creator4/2  "Cbar"
  S/1 -> Bus Creator4/1  "S"
  TriggerDamage/1(damagecase) -> [DamageCase]
  Inertia/Mass/CG Shift/1(Inertia) -> Demux/1
  Surfaces/1 -> Bus Selector1/1
  Engines/1 -> Bus Selector/1
  Bus Creator4/1 -> AC_parameters/1

== system gtm_design_lpv/GTM_T2/Actuators ==
  cmds : Inport
  Acutator Dynamics : Subsystem
  Acutator Dynamics (Unbiased) : Subsystem  Commented=on
  DeadBand : Subsystem
  InputModification for Trimming : Subsystem
  Label : Subsystem
  TimeDelay with IC feedthrough : Subsystem
  Surface Pos : Outport
  wires:
  TimeDelay with IC feedthrough/1(O) -> InputModification for Trimming/1(CmdVec)
  DeadBand/1(O) -> Surface Pos/1
  cmds/1 -> Acutator Dynamics/1(In)
  [SurfaceDeltas] -> InputModification for Trimming/3(SurfaceDeltas)
  Label/1(O) -> DeadBand/1(I)
  [SurfaceBias] -> InputModification for Trimming/2(SurfBias)
  InputModification for Trimming/1(CmdVecOut) -> Label/1(I)
  Acutator Dynamics/1(Out) -> TimeDelay with IC feedthrough/1(I)

== system gtm_design_lpv/GTM_T2/Aero ==
  Surfaces : Inport
  AuxVars : Inport  Port=2
  State : Inport  Port=3
  Basic Airframe : Subsystem
  Bus Selector1 : BusSelector  OutputSignals=CG,CP
  Bus Selector2 : BusSelector  OutputSignals=alpha,beta
  Bus Selector3 : BusSelector  OutputSignals=alpha  OutputAsBus=on
  Bus Selector4 : BusSelector  OutputSignals=beta  OutputAsBus=on
  Bus Selector6 : BusSelector  OutputSignals=tas
  Bus Selector7 : BusSelector  OutputSignals=qbar
  Bus Selector8 : BusSelector  OutputSignals=pb,qb,rb  OutputAsBus=on
  Bus to Vector5 : BusToVector
  Coefficent Evaluation : Subsystem  mask{b=b, cbar=Cbar, Sref=S}
      mask prompts: b "Reference Span (b)"; cbar "Reference Chord (cbar)"; Sref "Reference Area (Sref)"
      mask help:
      | Calulates the Force and Moments due to aerodynamic loads from vector of body axes aerodynamic coefficients:
      |    C6body = [Cx Cy Cz Cl Cm Cn].
      | Also requires dynamic pressure, cg/cp locations and reference lengths/area.
  Control Surfaces : Subsystem
  Dynamic Derviatives : Subsystem
  Label : Subsystem
  Stall Rolling Moment Asymmetry : Subsystem
  Sum8 : Sum  Inputs=++++  InputSameDT=on  SaturateOnIntegerOverflow=on  OutDataTypeStr=Inherit: Same as first input
  stall_cl_asym_enabled : Constant  Value=stall_cl_asym_enabled
  symmetry_on : Constant  Value=symmetric_aero_on
  FM : Outport
  Aero : Outport  Port=2
  wires:
  [AC_Params] -> Dynamic Derviatives/5(AC_Params)
  Bus to Vector5/1 -> Dynamic Derviatives/4(pqr)
  Bus Selector6/1 -> Dynamic Derviatives/3(TAS)  "<tas>"
  [AC_Params] -> Basic Airframe/4(AC_Params)
  Bus Selector8/1 -> Bus to Vector5/1  "pqr"
  Basic Airframe/1(C6) -> Sum8/1
  Control Surfaces/1(dC6) -> Sum8/2
  Dynamic Derviatives/1(dC6) -> Sum8/3
  State/1 -> Bus Selector8/1
  Bus Selector2/2 -> Basic Airframe/2(beta), Dynamic Derviatives/2(beta), Control Surfaces/2(beta)  "<beta>"
  Bus Selector2/1 -> Basic Airframe/1(alpha), Control Surfaces/1(alpha), Dynamic Derviatives/1(alpha)  "<alpha>"
  AuxVars/1 -> Bus Selector2/1, Bus Selector6/1, Bus Selector3/1, Bus Selector7/1, Bus Selector4/1
  Label/1(O) -> FM/1
  Bus Selector7/1 -> Coefficent Evaluation/2(qbar)  "<qbar>"
  Sum8/1 -> Aero/1, Coefficent Evaluation/1(C6 Body)
  Coefficent Evaluation/1(Forces) -> Label/1(If)
  Coefficent Evaluation/2(Moments) -> Label/2(Im)
  Bus Selector1/1 -> Coefficent Evaluation/3(Cg)  "<CG>"
  [AC_Params] -> Bus Selector1/1
  Bus Selector1/2 -> Coefficent Evaluation/4(Cp)  "<CP>"
  symmetry_on/1 -> Basic Airframe/3(symmetry_on)
  Surfaces/1 -> Control Surfaces/3(surfaces)
  stall_cl_asym_enabled/1 -> Stall Rolling Moment Asymmetry/3(stall_cl_asym_enabled)
  Stall Rolling Moment Asymmetry/1(dC6) -> Sum8/4
  Bus Selector3/1 -> Stall Rolling Moment Asymmetry/1(alpha)
  Bus Selector4/1 -> Stall Rolling Moment Asymmetry/2(beta)
  [AC_Params] -> Control Surfaces/4(AC_Params)

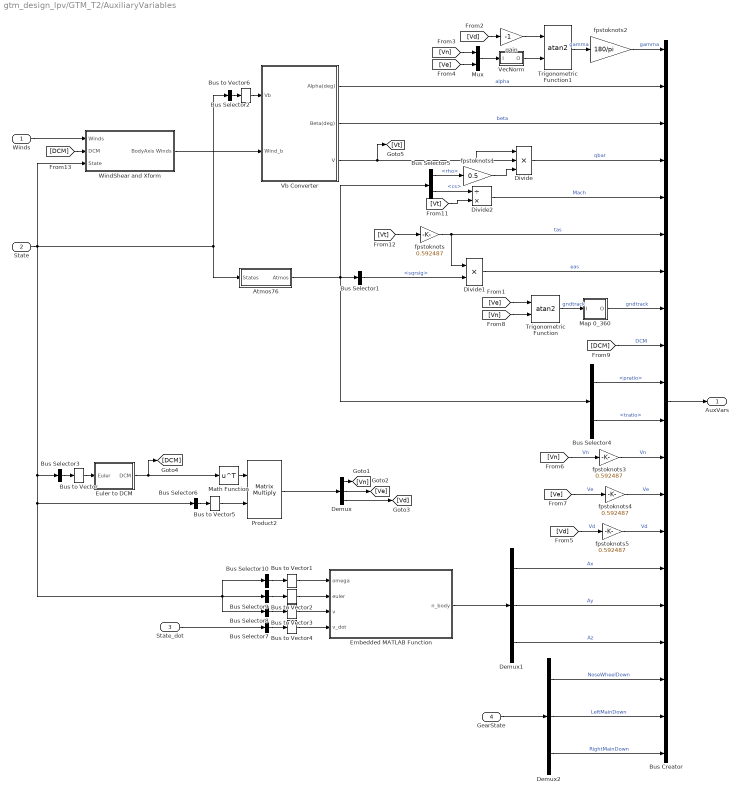
== system gtm_design_lpv/GTM_T2/AuxiliaryVariables ==
  Winds : Inport  PortDimensions=6
  State : Inport  Port=2
  State_dot : Inport  Port=3
  GearState : Inport  Port=4
  Atmos76 : Subsystem
  Bus Creator : BusCreator  Inputs=20
  Bus Selector1 : BusSelector  OutputSignals=sqrsig
  Bus Selector10 : BusSelector  OutputSignals=pb,qb,rb  OutputAsBus=on
  Bus Selector2 : BusSelector  OutputSignals=ub,vb,wb  OutputAsBus=on
  Bus Selector3 : BusSelector  OutputSignals=phi,theta,psi  OutputAsBus=on
  Bus Selector4 : BusSelector  OutputSignals=pratio,tratio
  Bus Selector5 : BusSelector  OutputSignals=rho,cs
  Bus Selector6 : BusSelector  OutputSignals=ub,vb,wb  OutputAsBus=on
  Bus Selector7 : BusSelector  OutputSignals=ub_dot,vb_dot,wb_dot  OutputAsBus=on
  Bus Selector8 : BusSelector  OutputSignals=ub,vb,wb  OutputAsBus=on
  Bus Selector9 : BusSelector  OutputSignals=phi,theta,psi  OutputAsBus=on
  Bus to Vector{,1..6} (7 alike) : BusToVector
  Demux : Demux  Outputs=3
  Demux1 : Demux  Outputs=3
  Demux2 : Demux  Outputs=3
  Divide : Product  Inputs=***
  Divide1 : Product
  Divide2 : Product  Inputs=/*
  Embedded MATLAB Function : MATLAB Function  TreatAsAtomicUnit=on
  Euler to DCM : Subsystem
  Map 0_360 : Subsystem
  Math Function : Math  Operator=transpose  SignedPower=on  SaturateOnIntegerOverflow=on
  Mux : Mux  Inputs=2
  Product2 : Product  Multiplication=Matrix(*)  RndMeth=Zero
  Trigonometric Function : Trigonometry  Operator=atan2
  Trigonometric Function1 : Trigonometry  Operator=atan2
  Vb Converter : Subsystem
  VecNorm : Subsystem
  WindShear and Xform : Subsystem
  fpstoknots{,3..5} (4 alike) : Gain  Gain=0.592487
  fpstoknots1 : Gain  Gain=0.5
  fpstoknots2 : Gain  Gain=180/pi
  gain : Gain  Gain=-1
  AuxVars : Outport
  wires:
  Demux2/3 -> Bus Creator/20  "RightMainDown"
  Demux2/2 -> Bus Creator/19  "LeftMainDown"
  Demux2/1 -> Bus Creator/18  "NoseWheelDown"
  GearState/1 -> Demux2/1
  [DCM] -> WindShear and Xform/2(DCM)
  WindShear and Xform/1(BodyAxis Winds) -> Vb Converter/2(Wind_b)
  Winds/1 -> WindShear and Xform/1(Winds)
  Product2/1 -> Demux/1
  Bus to Vector6/1 -> Vb Converter/1(Vb)
  Bus Selector2/1 -> Bus to Vector6/1
  Bus to Vector5/1 -> Product2/2
  Bus to Vector4/1 -> Embedded MATLAB Function/4(v_dot)
  Bus to Vector3/1 -> Embedded MATLAB Function/3(v)
  Bus to Vector2/1 -> Embedded MATLAB Function/2(euler)
  Bus to Vector1/1 -> Embedded MATLAB Function/1(omega)
  Bus to Vector/1 -> Euler to DCM/1("Euler ")
  Bus Selector3/1 -> Bus to Vector/1
  Bus Selector6/1 -> Bus to Vector5/1
  Math Function/1 -> Product2/1
  Demux/1 -> [Vn]
  Demux/2 -> [Ve]
  Embedded MATLAB Function/1(n_body) -> Demux1/1
  Demux1/3 -> Bus Creator/17  "Az"
  Demux1/2 -> Bus Creator/16  "Ay"
  Demux1/1 -> Bus Creator/15  "Ax"
  Bus Selector10/1 -> Bus to Vector1/1
  Bus Selector9/1 -> Bus to Vector2/1
  Bus Selector8/1 -> Bus to Vector3/1
  State_dot/1 -> Bus Selector7/1
  Bus Selector7/1 -> Bus to Vector4/1
  Bus Creator/1 -> AuxVars/1
  [Vt] -> fpstoknots/1
  [Vt] -> Divide2/2
  [DCM] -> Bus Creator/9  "DCM"
  fpstoknots5/1 -> Bus Creator/14  "Vd"
  fpstoknots4/1 -> Bus Creator/13  "Ve"
  fpstoknots3/1 -> Bus Creator/12  "Vn"
  Divide2/1 -> Bus Creator/5  "Mach"
  Bus Selector5/2 -> Divide2/1  "<cs>"
  Trigonometric Function/1 -> Map 0_360/1(I)  "gndtrack"
  Map 0_360/1(O) -> Bus Creator/8  "gndtrack"
  [Vn] -> Trigonometric Function/2
  [Ve] -> Trigonometric Function/1
  Bus Selector4/2 -> Bus Creator/11  "<tratio>"
  Bus Selector4/1 -> Bus Creator/10  "<pratio>"
  [Vd] -> fpstoknots5/1  "Vd"
  [Vn] -> fpstoknots3/1  "Vn"
  [Ve] -> fpstoknots4/1  "Ve"
  Divide1/1 -> Bus Creator/7  "eas"
  State/1 -> WindShear and Xform/3(State), Bus Selector3/1, Bus Selector6/1, Bus Selector8/1, Bus Selector10/1, Bus Selector9/1, Atmos76/1(States), Bus Selector2/1
  Atmos76/1(Atmos) -> Bus Selector4/1, Bus Selector1/1, Bus Selector5/1
  fpstoknots/1 -> Bus Creator/6, Divide1/1  "tas"
  Vb Converter/3(V) -> [Vt], Divide/1, Divide/2
  Bus Selector1/1 -> Divide1/2  "<sqrsig>"
  Vb Converter/1(Alpha(deg)) -> Bus Creator/2  "alpha"
  Vb Converter/2(Beta(deg)) -> Bus Creator/3  "beta"
  Bus Selector5/1 -> fpstoknots1/1  "<rho>"
  fpstoknots1/1 -> Divide/3
  Divide/1 -> Bus Creator/4  "qbar"
  Euler to DCM/1(DCM) -> Math Function/1, [DCM]
  Demux/3 -> [Vd]
  Trigonometric Function1/1 -> fpstoknots2/1  "gamma"
  gain/1 -> Trigonometric Function1/1
  [Vd] -> gain/1
  Mux/1 -> VecNorm/1(I)
  [Vn] -> Mux/1
  [Ve] -> Mux/2
  VecNorm/1(O) -> Trigonometric Function1/2
  fpstoknots2/1 -> Bus Creator/1  "gamma"

== system gtm_design_lpv/GTM_T2/EOM ==
  ThrustFM : Inport
  AeroFM : Inport  Port=2
  GravityFM : Inport  Port=3
  GearFM : Inport  Port=4
  AC_Params : Inport  Port=5
  Add : Sum  Inputs=++++
  Aircraft 6DOF : Subsystem  mask{UnitOfLength=ft}
      mask prompts: UnitOfLength "Length Unit"
      mask help:
      | Six Degree of Freedom Aircraft Simulation
      |
      | Input forces are both linear forces and torques -> [Fx Fy Fz Tl Tm Tn].
      | Inertia6 is a vector [Ixx Iyy Izz  Ixz Iyz Ixy], all positive
      | State Vector is [Vb pqr LatLonAlt PhiThetaPsi]
      mask init:
      | if (UnitOfLength==1), % ft
      |     Re=6.37043246e+06/.3048;
      | elseif (UnitOfLength==2), % m
      |     Re=6.37043246e+06;
      | end
      mask TypeOptions UnitOfLength: ft | meters
  Anti Windup : Subsystem
  Bus Selector1 : BusSelector  OutputSignals=Ixx,Iyy,Izz,Ixz,Iyz,Ixy  OutputAsBus=on
  Bus Selector11 : BusSelector  OutputSignals=mass
  Bus to Vector : BusToVector
  Bus to Vector1 : BusToVector
  Bus to Vector2 : BusToVector
  Integrator : Integrator  InitialCondition=StatesInp
  State Labels : Subsystem
  Xdot Labels : Subsystem
  State : Outport
  StateDeriv : Outport  Port=2
  wires:
  Bus to Vector2/1 -> Add/2
  Bus to Vector1/1 -> Add/1
  ThrustFM/1 -> Bus to Vector1/1
  AeroFM/1 -> Bus to Vector2/1
  State Labels/1(O) -> State/1
  Bus to Vector/1 -> Aircraft 6DOF/3(Inertia6)
  GearFM/1 -> Add/4
  GravityFM/1 -> Add/3
  Add/1 -> Aircraft 6DOF/1(Forces)
  Xdot Labels/1(O) -> StateDeriv/1
  Bus Selector1/1 -> Bus to Vector/1
  Aircraft 6DOF/1(Xdot) -> Xdot Labels/1(I), Integrator/1
  Anti Windup/1(O) -> State Labels/1(I)
  Integrator/1 -> Aircraft 6DOF/4(State), Anti Windup/1(I)
  Bus Selector11/1 -> Aircraft 6DOF/2(mass)  "<mass>"
  AC_Params/1 -> Bus Selector1/1, Bus Selector11/1
